simulink model "BEV_Thermal_Management"  (R2025a)
settings: Solver=ode23t  StartTime=0  StopTime=765  MaxStep=5  RelTol=1e-3  AbsTol=1e-3
model workspace: external: MATLAB File BEV_Thermal_Management_param.m (data not in the file)
undefined symbols (not defined in the file): Battery, bulb, cabin_doors_conductivity, cabin_duct_area, cabin_glass_conductivity, cabin_roof_conductivity, cabin_T_init, chiller_area_primary, chiller_N_baffles, chiller_N_tubes, chiller_tube_D, chiller_tube_L, chiller_wall_conductivity, chiller_wall_thickness, compressor_rpm_LUT, condenser_air_area_flow, condenser_air_area_primary, condenser_W, condenser_wall_conductivity, condenser_wall_thickness, coolant_channel_D, coolant_pipe_area, coolant_pipe_D, coolant_T_init, coolant_tank_area, coolant_tank_volume, coolant_valve_D_ratio_max, coolant_valve_D_ratio_min, coolant_valve_displacement, coolant_valve_S_max, cycle, DCDC, Edrive, evaporator_air_area_flow, evaporator_air_area_primary, evaporator_W, evaporator_wall_conductivity, evaporator_wall_thickness, heater_max_power, ModuleType1, outlet, ptc_max_power, pump_speed_max, radiationReflectionShields, radiator_air_area_flow, radiator_air_area_primary, radiator_W, radiator_wall_conductivity, radiator_wall_thickness, refrigerant_alpha_init, refrigerant_pipe_D, transRatio
libraries: fl_lib x264, nesl_utility x91, SimscapeFluids_lib x22, sdl_lib x13, ee_lib x9, nesl_utility_internal x4, slpidlib x3, BatteryProtection x3, batt_lib x2, BatteryCurrentManagement x1, autolibsharedcommon x1, simulink x1
(part 8 of 9)

== system BEV_Thermal_Management/Evaporator/SR5 ==
  Absolute Reference (2P) : fl_lib/Two-Phase Fluid/Elements/Absolute Reference (2P)
  Mass & Energy Flow Rate Sensor (2P) : fl_lib/Two-Phase Fluid/Sensors/Flow Rate Sensor (2P)  mass_flow_measure=true  volumetric_flow_measure=false  energy_flow_measure=true
      settings: InternalSimscapePortConfiguration="{\"Bottom\":[{\"id\":\"PHI\",\"label\":\"φ\",\"type\":\"output\"}],\"Left\":[{\"id\":\"A\",\"label\":\"A\",\"type\":\"foundation.two_phase_fluid.two_phase_fluid\"}],\"Right\":[{\"id\":\"B\",\"label\":\"B\",\"type\":\"foundation.two_phase_fluid.two_phase_fluid\"},{\"id\":\"M\",\"label\":\"M\",\"type\":\"output\"}],\"Top\":[]}"
  PS-Simulink Converter : nesl_utility/PS-Simulink Converter  PhysicalDomain=network_engine_domain  SubClassName=ps_output  LeftPortType=input  RightPortType=output  PseudoPeriodic=off  Frequencies=[]  VectorFormat=1-D array  Unit=W  AffineConversion=off
  PS-Simulink Converter1 : nesl_utility/PS-Simulink Converter  PhysicalDomain=network_engine_domain  SubClassName=ps_output  LeftPortType=input  RightPortType=output  PseudoPeriodic=off  Frequencies=[]  VectorFormat=inherit  Unit=degC  AffineConversion=off
  Pressure & Internal Energy Sensor (2P) : fl_lib/Two-Phase Fluid/Sensors/Pressure, Temperature & Internal Energy Sensor (2P)  reference=foundation.enum.MeasurementReference.difference  pressure=true  pressure_spec=foundation.enum.PressureMeasementSpec.Absolute  temperature=false  internal_energy=true
      settings: InternalSimscapePortConfiguration="{\"Bottom\":[{\"id\":\"U\",\"label\":\"U\",\"type\":\"output\"}],\"Left\":[{\"id\":\"A\",\"label\":\"A\",\"type\":\"foundation.two_phase_fluid.two_phase_fluid\"}],\"Right\":[{\"id\":\"B\",\"label\":\"B\",\"type\":\"foundation.two_phase_fluid.two_phase_fluid\"},{\"id\":\"P\",\"label\":\"P\",\"type\":\"output\"}],\"Top\":[]}"
  Terminator : Terminator
  Thermodynamic Properties Sensor (2P)1 : fl_lib/Two-Phase Fluid/Sensors/Thermodynamic Properties Sensor (2P)  temperature=true  enthalpy=true  density=false  specific_volume=true  entropy=true
      settings: InternalSimscapePortConfiguration="{\"Bottom\":[{\"id\":\"V\",\"label\":\"v\",\"type\":\"output\"},{\"id\":\"S\",\"label\":\"s\",\"type\":\"output\"}],\"Left\":[{\"id\":\"A\",\"label\":\"A\",\"type\":\"foundation.two_phase_fluid.two_phase_fluid\"}],\"Right\":[{\"id\":\"T\",\"label\":\"T\",\"type\":\"output\"},{\"id\":\"H\",\"label\":\"h\",\"type\":\"output\"}],\"Top\":[]}"
  B : PMIOPort  Side=Left
  A : PMIOPort  Port=2  Side=Right
  tag scope: Phi_evap_in=global
  wires:
  PS-Simulink Converter/1 -> [Phi_evap_in]
  PS-Simulink Converter1/1 -> Terminator/1  "tempRefEvapIn"
  connections:
  B/RConn1 -- Mass & Energy Flow Rate Sensor (2P)/RConn1
  Mass & Energy Flow Rate Sensor (2P)/LConn1 -- Thermodynamic Properties Sensor (2P)1/LConn1 -- Pressure & Internal Energy Sensor (2P)/LConn1 -- A/RConn1
  Mass & Energy Flow Rate Sensor (2P)/RConn3 -- PS-Simulink Converter/LConn1
  Absolute Reference (2P)/LConn1 -- Pressure & Internal Energy Sensor (2P)/RConn1
  PS-Simulink Converter1/LConn1 -- Thermodynamic Properties Sensor (2P)1/RConn1

== system BEV_Thermal_Management/Evaporator/SR6 ==
  Absolute Reference (2P) : fl_lib/Two-Phase Fluid/Elements/Absolute Reference (2P)
  Mass & Energy Flow Rate Sensor (2P) : fl_lib/Two-Phase Fluid/Sensors/Flow Rate Sensor (2P)  mass_flow_measure=true  volumetric_flow_measure=false  energy_flow_measure=true
      settings: InternalSimscapePortConfiguration="{\"Bottom\":[{\"id\":\"PHI\",\"label\":\"φ\",\"type\":\"output\"}],\"Left\":[{\"id\":\"A\",\"label\":\"A\",\"type\":\"foundation.two_phase_fluid.two_phase_fluid\"}],\"Right\":[{\"id\":\"B\",\"label\":\"B\",\"type\":\"foundation.two_phase_fluid.two_phase_fluid\"},{\"id\":\"M\",\"label\":\"M\",\"type\":\"output\"}],\"Top\":[]}"
  PS-Simulink Converter : nesl_utility/PS-Simulink Converter  PhysicalDomain=network_engine_domain  SubClassName=ps_output  LeftPortType=input  RightPortType=output  PseudoPeriodic=off  Frequencies=[]  VectorFormat=1-D array  Unit=W  AffineConversion=off
  PS-Simulink Converter1 : nesl_utility/PS-Simulink Converter  PhysicalDomain=network_engine_domain  SubClassName=ps_output  LeftPortType=input  RightPortType=output  PseudoPeriodic=off  Frequencies=[]  VectorFormat=1-D array  Unit=MPa  AffineConversion=off
  PS-Simulink Converter2 : nesl_utility/PS-Simulink Converter  PhysicalDomain=network_engine_domain  SubClassName=ps_output  LeftPortType=input  RightPortType=output  PseudoPeriodic=off  Frequencies=[]  VectorFormat=inherit  Unit=degC  AffineConversion=off
  Pressure & Internal Energy Sensor (2P) : fl_lib/Two-Phase Fluid/Sensors/Pressure, Temperature & Internal Energy Sensor (2P)  reference=foundation.enum.MeasurementReference.difference  pressure=true  pressure_spec=foundation.enum.PressureMeasementSpec.Absolute  temperature=false  internal_energy=true
      settings: InternalSimscapePortConfiguration="{\"Bottom\":[{\"id\":\"U\",\"label\":\"U\",\"type\":\"output\"}],\"Left\":[{\"id\":\"A\",\"label\":\"A\",\"type\":\"foundation.two_phase_fluid.two_phase_fluid\"}],\"Right\":[{\"id\":\"B\",\"label\":\"B\",\"type\":\"foundation.two_phase_fluid.two_phase_fluid\"},{\"id\":\"P\",\"label\":\"P\",\"type\":\"output\"}],\"Top\":[]}"
  Terminator : Terminator
  Thermodynamic Properties Sensor (2P)1 : fl_lib/Two-Phase Fluid/Sensors/Thermodynamic Properties Sensor (2P)  temperature=true  enthalpy=true  density=false  specific_volume=true  entropy=true
      settings: InternalSimscapePortConfiguration="{\"Bottom\":[{\"id\":\"V\",\"label\":\"v\",\"type\":\"output\"},{\"id\":\"S\",\"label\":\"s\",\"type\":\"output\"}],\"Left\":[{\"id\":\"A\",\"label\":\"A\",\"type\":\"foundation.two_phase_fluid.two_phase_fluid\"}],\"Right\":[{\"id\":\"T\",\"label\":\"T\",\"type\":\"output\"},{\"id\":\"H\",\"label\":\"h\",\"type\":\"output\"}],\"Top\":[]}"
  B : PMIOPort  Side=Left
  A : PMIOPort  Port=2  Side=Right
  tag scope: Phi_evap_out=global, p_evap=global
  wires:
  PS-Simulink Converter/1 -> [Phi_evap_out]
  PS-Simulink Converter1/1 -> [p_evap]
  PS-Simulink Converter2/1 -> Terminator/1  "tempRefEvapOut"
  connections:
  B/RConn1 -- Mass & Energy Flow Rate Sensor (2P)/RConn1
  Mass & Energy Flow Rate Sensor (2P)/LConn1 -- Thermodynamic Properties Sensor (2P)1/LConn1 -- Pressure & Internal Energy Sensor (2P)/LConn1 -- A/RConn1
  Mass & Energy Flow Rate Sensor (2P)/RConn3 -- PS-Simulink Converter/LConn1
  Absolute Reference (2P)/LConn1 -- Pressure & Internal Energy Sensor (2P)/RConn1
  PS-Simulink Converter1/LConn1 -- Pressure & Internal Energy Sensor (2P)/RConn2
  PS-Simulink Converter2/LConn1 -- Thermodynamic Properties Sensor (2P)1/RConn1

== system BEV_Thermal_Management/Heater/Current calculator ==
  Controlled Current Source : fl_lib/Electrical/Electrical Sources/Controlled Current Source
  Electrical Reference : fl_lib/Electrical/Electrical Elements/Electrical Reference
  Electrical Reference1 : fl_lib/Electrical/Electrical Elements/Electrical Reference
  PS Divide : fl_lib/Physical Signals/Functions/PS Divide
  Voltage Sensor : fl_lib/Electrical/Electrical Sensors/Voltage Sensor
  Conn2 : PMIOPort  Side=Left
  Conn1 : PMIOPort  Port=2  Side=Left
  connections:
  Electrical Reference/LConn1 -- Controlled Current Source/LConn1
  Controlled Current Source/RConn2 -- Voltage Sensor/LConn1 -- Conn2/RConn1
  PS Divide/LConn1 -- Conn1/RConn1
  Voltage Sensor/RConn2 -- Electrical Reference1/LConn1
  Controlled Current Source/RConn1 -- PS Divide/RConn1
  Voltage Sensor/RConn1 -- PS Divide/LConn2

== system BEV_Thermal_Management/Heater/SC1 ==
  Absolute Reference (TL) : fl_lib/Thermal Liquid/Elements/Absolute Reference (TL)
  PS-Simulink Converter1 : nesl_utility/PS-Simulink Converter  PhysicalDomain=network_engine_domain  SubClassName=ps_output  LeftPortType=input  RightPortType=output  PseudoPeriodic=off  Frequencies=[]  VectorFormat=inherit  Unit=degC  AffineConversion=on
  Pressure & Temperature Sensor (TL) : fl_lib/Thermal Liquid/Sensors/Pressure & Temperature Sensor (TL)  reference=foundation.enum.MeasurementReference.difference  pressure=true  pressure_spec=foundation.enum.PressureMeasementSpec.Absolute  temperature=true
      settings: InternalSimscapePortConfiguration="{\"Bottom\":[{\"id\":\"T\",\"label\":\"T\",\"type\":\"output\"}],\"Left\":[{\"id\":\"A\",\"label\":\"A\",\"type\":\"foundation.thermal_liquid.thermal_liquid\"}],\"Right\":[{\"id\":\"B\",\"label\":\"B\",\"type\":\"foundation.thermal_liquid.thermal_liquid\"},{\"id\":\"P\",\"label\":\"P\",\"type\":\"output\"}],\"Top\":[]}"
  Terminator : Terminator
  B : PMIOPort  Side=Left
  A : PMIOPort  Port=2  Side=Right
  wires:
  PS-Simulink Converter1/1 -> Terminator/1  "tempCoolHeaterOut"
  connections:
  Pressure & Temperature Sensor (TL)/LConn1 -- A/RConn1 -- B/RConn1
  Absolute Reference (TL)/LConn1 -- Pressure & Temperature Sensor (TL)/RConn1
  PS-Simulink Converter1/LConn1 -- Pressure & Temperature Sensor (TL)/RConn3

== system BEV_Thermal_Management/Heater/SC7 ==
  Absolute Reference (TL) : fl_lib/Thermal Liquid/Elements/Absolute Reference (TL)
  PS-Simulink Converter1 : nesl_utility/PS-Simulink Converter  PhysicalDomain=network_engine_domain  SubClassName=ps_output  LeftPortType=input  RightPortType=output  PseudoPeriodic=off  Frequencies=[]  VectorFormat=inherit  Unit=degC  AffineConversion=on
  Pressure & Temperature Sensor (TL) : fl_lib/Thermal Liquid/Sensors/Pressure & Temperature Sensor (TL)  reference=foundation.enum.MeasurementReference.difference  pressure=true  pressure_spec=foundation.enum.PressureMeasementSpec.Absolute  temperature=true
      settings: InternalSimscapePortConfiguration="{\"Bottom\":[{\"id\":\"T\",\"label\":\"T\",\"type\":\"output\"}],\"Left\":[{\"id\":\"A\",\"label\":\"A\",\"type\":\"foundation.thermal_liquid.thermal_liquid\"}],\"Right\":[{\"id\":\"B\",\"label\":\"B\",\"type\":\"foundation.thermal_liquid.thermal_liquid\"},{\"id\":\"P\",\"label\":\"P\",\"type\":\"output\"}],\"Top\":[]}"
  Terminator : Terminator
  B : PMIOPort  Side=Left
  A : PMIOPort  Port=2  Side=Right
  wires:
  PS-Simulink Converter1/1 -> Terminator/1  "tempCoolHeaterIn"
  connections:
  Pressure & Temperature Sensor (TL)/LConn1 -- A/RConn1 -- B/RConn1
  Absolute Reference (TL)/LConn1 -- Pressure & Temperature Sensor (TL)/RConn1
  PS-Simulink Converter1/LConn1 -- Pressure & Temperature Sensor (TL)/RConn3

== system BEV_Thermal_Management/Motor/PWRS3 ==
  Electrical Reference : fl_lib/Electrical/Electrical Elements/Electrical Reference
  PS Terminator : fl_lib/Physical Signals/Sinks/PS Terminator
  Power Sensor : ee_lib/Sensors & Transducers/Power Sensor  measurement_type=1  averaging_period=1e-4 s
  HV : PMIOPort  Side=Left
  EM : PMIOPort  Port=2  Side=Right
  connections:
  Power Sensor/LConn1 -- HV/RConn1
  Power Sensor/LConn2 -- EM/RConn1
  Power Sensor/LConn3 -- Electrical Reference/LConn1
  PS Terminator/LConn1 -- Power Sensor/RConn1

== system BEV_Thermal_Management/Motor/PWRS4 ==
  Mechanical Rotational Reference : fl_lib/Mechanical/Rotational Elements/Mechanical Rotational Reference
  PS Terminator : fl_lib/Physical Signals/Sinks/PS Terminator
  Power : sdl_lib/Sensors/Rotational Power Sensor  measurement_type=sdl.enum.rotationalPowerSensorType.instantaneous  averaging_period=1 s  max_frequency=1000 Hz  max_speed=1000 rpm
      settings: InternalSimscapePortConfiguration="{\"Bottom\":[],\"Left\":[{\"id\":\"S\",\"label\":\"S\",\"type\":\"foundation.mechanical.rotational.rotational\"},{\"id\":\"R\",\"label\":\"R\",\"type\":\"foundation.mechanical.rotational.rotational\"},{\"id\":\"C\",\"label\":\"C\",\"type\":\"foundation.mechanical.rotational.rotational\"}],\"Right\":[{\"id\":\"P\",\"label\":\"P\",\"type\":\"output\"}],\"Top\":[]}"
  C : PMIOPort  Side=Left
  B : PMIOPort  Port=2  Side=Right
  connections:
  Power/LConn1 -- C/RConn1
  Power/LConn3 -- Mechanical Rotational Reference/LConn1
  B/RConn1 -- Power/LConn2
  Power/RConn1 -- PS Terminator/LConn1

== system BEV_Thermal_Management/Motor/PWRS5 ==
  Mechanical Rotational Reference : fl_lib/Mechanical/Rotational Elements/Mechanical Rotational Reference
  PS Terminator : fl_lib/Physical Signals/Sinks/PS Terminator
  Power : sdl_lib/Sensors/Rotational Power Sensor  measurement_type=sdl.enum.rotationalPowerSensorType.instantaneous  averaging_period=1 s  max_frequency=1000 Hz  max_speed=1000 rpm
      settings: InternalSimscapePortConfiguration="{\"Bottom\":[],\"Left\":[{\"id\":\"S\",\"label\":\"S\",\"type\":\"foundation.mechanical.rotational.rotational\"},{\"id\":\"R\",\"label\":\"R\",\"type\":\"foundation.mechanical.rotational.rotational\"},{\"id\":\"C\",\"label\":\"C\",\"type\":\"foundation.mechanical.rotational.rotational\"}],\"Right\":[{\"id\":\"P\",\"label\":\"P\",\"type\":\"output\"}],\"Top\":[]}"
  F : PMIOPort  Side=Left
  RA : PMIOPort  Port=2  Side=Right
  connections:
  Power/LConn1 -- F/RConn1
  Power/LConn3 -- Mechanical Rotational Reference/LConn1
  RA/RConn1 -- Power/LConn2
  Power/RConn1 -- PS Terminator/LConn1

== system BEV_Thermal_Management/Motor/SC5 ==
  Absolute Reference (TL) : fl_lib/Thermal Liquid/Elements/Absolute Reference (TL)
  Mass & Energy Flow Rate Sensor (TL) : fl_lib/Thermal Liquid/Sensors/Flow Rate Sensor (TL)  mass_flow_measure=true  volumetric_flow_measure=false  energy_flow_measure=true
      settings: InternalSimscapePortConfiguration="{\"Bottom\":[{\"id\":\"PHI\",\"label\":\"φ\",\"type\":\"output\"}],\"Left\":[{\"id\":\"A\",\"label\":\"A\",\"type\":\"foundation.thermal_liquid.thermal_liquid\"}],\"Right\":[{\"id\":\"B\",\"label\":\"B\",\"type\":\"foundation.thermal_liquid.thermal_liquid\"},{\"id\":\"M\",\"label\":\"M\",\"type\":\"output\"}],\"Top\":[]}"
  PS-Simulink Converter : nesl_utility/PS-Simulink Converter  PhysicalDomain=network_engine_domain  SubClassName=ps_output  LeftPortType=input  RightPortType=output  PseudoPeriodic=off  Frequencies=[]  VectorFormat=1-D array  Unit=W  AffineConversion=off
  PS-Simulink Converter1 : nesl_utility/PS-Simulink Converter  PhysicalDomain=network_engine_domain  SubClassName=ps_output  LeftPortType=input  RightPortType=output  PseudoPeriodic=off  Frequencies=[]  VectorFormat=inherit  Unit=degC  AffineConversion=on
  Pressure & Temperature Sensor (TL) : fl_lib/Thermal Liquid/Sensors/Pressure & Temperature Sensor (TL)  reference=foundation.enum.MeasurementReference.difference  pressure=true  pressure_spec=foundation.enum.PressureMeasementSpec.Absolute  temperature=true
      settings: InternalSimscapePortConfiguration="{\"Bottom\":[{\"id\":\"T\",\"label\":\"T\",\"type\":\"output\"}],\"Left\":[{\"id\":\"A\",\"label\":\"A\",\"type\":\"foundation.thermal_liquid.thermal_liquid\"}],\"Right\":[{\"id\":\"B\",\"label\":\"B\",\"type\":\"foundation.thermal_liquid.thermal_liquid\"},{\"id\":\"P\",\"label\":\"P\",\"type\":\"output\"}],\"Top\":[]}"
  Terminator : Terminator
  A : PMIOPort  Side=Left
  B : PMIOPort  Port=2  Side=Right
  tag scope: Phi_motor_in=global
  wires:
  PS-Simulink Converter/1 -> [Phi_motor_in]
  PS-Simulink Converter1/1 -> Terminator/1  "tempCoolEMIn"
  connections:
  Pressure & Temperature Sensor (TL)/LConn1 -- A/RConn1 -- Mass & Energy Flow Rate Sensor (TL)/LConn1
  Mass & Energy Flow Rate Sensor (TL)/RConn1 -- B/RConn1
  Absolute Reference (TL)/LConn1 -- Pressure & Temperature Sensor (TL)/RConn1
  Mass & Energy Flow Rate Sensor (TL)/RConn3 -- PS-Simulink Converter/LConn1
  PS-Simulink Converter1/LConn1 -- Pressure & Temperature Sensor (TL)/RConn3

== system BEV_Thermal_Management/Motor/SC6 ==
  Absolute Reference (TL) : fl_lib/Thermal Liquid/Elements/Absolute Reference (TL)
  Mass & Energy Flow Rate Sensor (TL) : fl_lib/Thermal Liquid/Sensors/Flow Rate Sensor (TL)  mass_flow_measure=true  volumetric_flow_measure=false  energy_flow_measure=true
      settings: InternalSimscapePortConfiguration="{\"Bottom\":[{\"id\":\"PHI\",\"label\":\"φ\",\"type\":\"output\"}],\"Left\":[{\"id\":\"A\",\"label\":\"A\",\"type\":\"foundation.thermal_liquid.thermal_liquid\"}],\"Right\":[{\"id\":\"B\",\"label\":\"B\",\"type\":\"foundation.thermal_liquid.thermal_liquid\"},{\"id\":\"M\",\"label\":\"M\",\"type\":\"output\"}],\"Top\":[]}"
  PS-Simulink Converter : nesl_utility/PS-Simulink Converter  PhysicalDomain=network_engine_domain  SubClassName=ps_output  LeftPortType=input  RightPortType=output  PseudoPeriodic=off  Frequencies=[]  VectorFormat=1-D array  Unit=W  AffineConversion=off
  PS-Simulink Converter1 : nesl_utility/PS-Simulink Converter  PhysicalDomain=network_engine_domain  SubClassName=ps_output  LeftPortType=input  RightPortType=output  PseudoPeriodic=off  Frequencies=[]  VectorFormat=1-D array  Unit=degC  AffineConversion=on
  PS-Simulink Converter2 : nesl_utility/PS-Simulink Converter  PhysicalDomain=network_engine_domain  SubClassName=ps_output  LeftPortType=input  RightPortType=output  PseudoPeriodic=off  Frequencies=[]  VectorFormat=inherit  Unit=kg/s  AffineConversion=off
  Pressure & Temperature Sensor (TL) : fl_lib/Thermal Liquid/Sensors/Pressure & Temperature Sensor (TL)  reference=foundation.enum.MeasurementReference.difference  pressure=true  pressure_spec=foundation.enum.PressureMeasementSpec.Absolute  temperature=true
      settings: InternalSimscapePortConfiguration="{\"Bottom\":[{\"id\":\"T\",\"label\":\"T\",\"type\":\"output\"}],\"Left\":[{\"id\":\"A\",\"label\":\"A\",\"type\":\"foundation.thermal_liquid.thermal_liquid\"}],\"Right\":[{\"id\":\"B\",\"label\":\"B\",\"type\":\"foundation.thermal_liquid.thermal_liquid\"},{\"id\":\"P\",\"label\":\"P\",\"type\":\"output\"}],\"Top\":[]}"
  Terminator : Terminator
  A : PMIOPort  Side=Left
  B : PMIOPort  Port=2  Side=Right
  tag scope: Phi_motor_out=global, T_coolant_motor_out=global
  wires:
  PS-Simulink Converter/1 -> [Phi_motor_out]
  PS-Simulink Converter1/1 -> [T_coolant_motor_out]  "tempCoolEMOut"
  PS-Simulink Converter2/1 -> Terminator/1  "tempCoolEMOut"
  connections:
  Pressure & Temperature Sensor (TL)/LConn1 -- A/RConn1 -- Mass & Energy Flow Rate Sensor (TL)/LConn1
  Mass & Energy Flow Rate Sensor (TL)/RConn1 -- B/RConn1
  Absolute Reference (TL)/LConn1 -- Pressure & Temperature Sensor (TL)/RConn1
  Mass & Energy Flow Rate Sensor (TL)/RConn3 -- PS-Simulink Converter/LConn1
  PS-Simulink Converter1/LConn1 -- Pressure & Temperature Sensor (TL)/RConn3
  PS-Simulink Converter2/LConn1 -- Mass & Energy Flow Rate Sensor (TL)/RConn2

== system BEV_Thermal_Management/Motor Pump/Power sensor ==
  MRR3 : fl_lib/Mechanical/Rotational Elements/Mechanical Rotational Reference
  Pump power : fl_lib/Physical Signals/Functions/PS Product
  Rotational Motion Sensor : fl_lib/Mechanical/Mechanical Sensors/Ideal Rotational Motion Sensor  reference=foundation.enum.MeasurementReference.difference  acceleration_port=false  velocity_port=true  position_port=true  wrap_angle=simscape.enum.onoff.off  offset=0 rad
  Torque Sensor : fl_lib/Mechanical/Mechanical Sensors/Ideal Torque Sensor
  A : PMIOPort  Side=Left
  P : PMIOPort  Port=2  Side=Left
  B : PMIOPort  Port=3  Side=Right
  connections:
  Torque Sensor/RConn2 -- Pump power/LConn1
  Torque Sensor/RConn1 -- B/RConn1
  Rotational Motion Sensor/LConn1 -- Torque Sensor/LConn1 -- A/RConn1
  Rotational Motion Sensor/RConn2 -- Pump power/LConn2
  MRR3/LConn1 -- Rotational Motion Sensor/RConn1
  Pump power/RConn1 -- P/RConn1

== system BEV_Thermal_Management/PTC/Current calculator ==
  Controlled Current Source : fl_lib/Electrical/Electrical Sources/Controlled Current Source
  Electrical Reference : fl_lib/Electrical/Electrical Elements/Electrical Reference
  Electrical Reference1 : fl_lib/Electrical/Electrical Elements/Electrical Reference
  PS Divide : fl_lib/Physical Signals/Functions/PS Divide
  Voltage Sensor : fl_lib/Electrical/Electrical Sensors/Voltage Sensor
  Conn2 : PMIOPort  Side=Left
  Conn1 : PMIOPort  Port=2  Side=Left
  connections:
  Electrical Reference/LConn1 -- Controlled Current Source/LConn1
  Controlled Current Source/RConn2 -- Conn2/RConn1 -- Voltage Sensor/LConn1
  PS Divide/LConn1 -- Conn1/RConn1
  Voltage Sensor/RConn2 -- Electrical Reference1/LConn1
  Controlled Current Source/RConn1 -- PS Divide/RConn1
  Voltage Sensor/RConn1 -- PS Divide/LConn2

== system BEV_Thermal_Management/Parallel-Serial Mode Valve/Battery Coolant Tank Heat Transfer ==
  Convective Heat Transfer : fl_lib/Thermal/Thermal Elements/Convective Heat Transfer  thermal_type=foundation.enum.constant_variable.constant  area=3 * coolant_tank_area m^2  heat_tr_coeff=20 W/(m^2 * K)  min_heat_tr_coeff=1e-3 W/(K*m^2)  T_specify=off  T_priority=None  T=0 K  T_nominal_specify=off  T_nominal_value=1  T_nominal_unit=K  Q_specify=off  Q_priority=None  Q=0 W  Q_nominal_specify=off  Q_nominal_value=1  Q_nominal_unit=W
  Convective Heat Transfer1 : fl_lib/Thermal/Thermal Elements/Convective Heat Transfer  thermal_type=foundation.enum.constant_variable.constant  area=3 * coolant_tank_area m^2  heat_tr_coeff=20 W/(m^2 * K)  min_heat_tr_coeff=1e-3 W/(K*m^2)  T_specify=off  T_priority=None  T=0 K  T_nominal_specify=off  T_nominal_value=1  T_nominal_unit=K  Q_specify=off  Q_priority=None  Q=0 W  Q_nominal_specify=off  Q_nominal_value=1  Q_nominal_unit=W
  Environment Temperature : fl_lib/Thermal/Thermal Sources/Controlled Temperature Source
  Simulink-PS Converter : nesl_utility/Simulink-PS Converter  PhysicalDomain=network_engine_domain  SubClassName=ps_input  LeftPortType=input  RightPortType=output  PseudoPeriodic=off  Frequencies=[]  NoiseDistribution=none  NoiseParameters=[]  Unit=degC  AffineConversion=on  FilteringAndDerivatives=provide  SimscapeFilterOrder=1  InputFilterTimeConstant=0.001  UdotUserProvided=0
  Thermal Reference : fl_lib/Thermal/Thermal Elements/Thermal Reference
  A : PMIOPort  Side=Left
  B : PMIOPort  Port=2  Side=Left
  wires:
  [T_env] -> Simulink-PS Converter/1
  connections:
  Environment Temperature/LConn1 -- Convective Heat Transfer/RConn1 -- Convective Heat Transfer1/RConn1
  Thermal Reference/LConn1 -- Environment Temperature/RConn2
  Simulink-PS Converter/RConn1 -- Environment Temperature/RConn1
  B/RConn1 -- Convective Heat Transfer1/LConn1
  Convective Heat Transfer/LConn1 -- A/RConn1

== system BEV_Thermal_Management/Parallel-Serial Mode Valve/Motor Coolant Tank Heat Transfer ==
  Convective Heat Transfer : fl_lib/Thermal/Thermal Elements/Convective Heat Transfer  thermal_type=foundation.enum.constant_variable.constant  area=3 * coolant_tank_area m^2  heat_tr_coeff=20 W/(m^2 * K)  min_heat_tr_coeff=1e-3 W/(K*m^2)  T_specify=off  T_priority=None  T=0 K  T_nominal_specify=off  T_nominal_value=1  T_nominal_unit=K  Q_specify=off  Q_priority=None  Q=0 W  Q_nominal_specify=off  Q_nominal_value=1  Q_nominal_unit=W
  Convective Heat Transfer1 : fl_lib/Thermal/Thermal Elements/Convective Heat Transfer  thermal_type=foundation.enum.constant_variable.constant  area=3 * coolant_tank_area m^2  heat_tr_coeff=20 W/(m^2 * K)  min_heat_tr_coeff=1e-3 W/(K*m^2)  T_specify=off  T_priority=None  T=0 K  T_nominal_specify=off  T_nominal_value=1  T_nominal_unit=K  Q_specify=off  Q_priority=None  Q=0 W  Q_nominal_specify=off  Q_nominal_value=1  Q_nominal_unit=W
  Environment Temperature : fl_lib/Thermal/Thermal Sources/Controlled Temperature Source
  Simulink-PS Converter : nesl_utility/Simulink-PS Converter  PhysicalDomain=network_engine_domain  SubClassName=ps_input  LeftPortType=input  RightPortType=output  PseudoPeriodic=off  Frequencies=[]  NoiseDistribution=none  NoiseParameters=[]  Unit=degC  AffineConversion=on  FilteringAndDerivatives=provide  SimscapeFilterOrder=1  InputFilterTimeConstant=0.001  UdotUserProvided=0
  Thermal Reference : fl_lib/Thermal/Thermal Elements/Thermal Reference
  A : PMIOPort  Side=Right
  B : PMIOPort  Port=2  Side=Right
  wires:
  [T_env] -> Simulink-PS Converter/1
  connections:
  Simulink-PS Converter/RConn1 -- Environment Temperature/RConn1
  Thermal Reference/LConn1 -- Environment Temperature/RConn2
  Convective Heat Transfer/RConn1 -- Environment Temperature/LConn1 -- Convective Heat Transfer1/RConn1
  B/RConn1 -- Convective Heat Transfer1/LConn1
  A/RConn1 -- Convective Heat Transfer/LConn1

== system BEV_Thermal_Management/Radiator/Ram Pressure ==
  1/2 : fl_lib/Physical Signals/Functions/PS Gain  gain=0.5
  Controlled Pressure Source (MA) : fl_lib/Moist Air/Sources/Pressure Source (MA)  source_type=foundation.enum.constant_controlled.controlled  pressure_differential=0 MPa  power_spec=foundation.enum.power_spec.isentropic  area_A=cabin_duct_area m^2  area_B=cabin_duct_area m^2
      settings: InternalSimscapePortConfiguration="{\"Bottom\":[],\"Left\":[{\"id\":\"A\",\"label\":\"A\",\"type\":\"foundation.moist_air.moist_air\"},{\"id\":\"P\",\"label\":\"P\",\"type\":\"input\"}],\"Right\":[{\"id\":\"B\",\"label\":\"B\",\"type\":\"foundation.moist_air.moist_air\"}],\"Top\":[]}"
  PS Product : fl_lib/Physical Signals/Functions/PS Product
  Thermodynamic Properties Sensor (MA) : fl_lib/Moist Air/Sensors/Thermodynamic Properties Sensor (MA)  measurement_mass_spec=foundation.enum.measurement_mass_spec.mixture  enthalpy=true  enthalpy_reference=foundation.enum.EnthalpyReference.PropertyTables  density=true  specific_heat=true  entropy=true
      settings: InternalSimscapePortConfiguration="{\"Bottom\":[{\"id\":\"CP\",\"label\":\"cp\",\"type\":\"output\"},{\"id\":\"S\",\"label\":\"s\",\"type\":\"output\"}],\"Left\":[{\"id\":\"A\",\"label\":\"A\",\"type\":\"foundation.moist_air.moist_air\"}],\"Right\":[{\"id\":\"H\",\"label\":\"h\",\"type\":\"output\"},{\"id\":\"RHO\",\"label\":\"ρ\",\"type\":\"output\"}],\"Top\":[]}"
  sqr : fl_lib/Physical Signals/Functions/PS Math Function  fcn_choice=foundation.enum.math_function.square  v=1
  A : PMIOPort  Side=Left
  V : PMIOPort  Port=2  Side=Left
  B : PMIOPort  Port=3  Side=Right
  connections:
  Controlled Pressure Source (MA)/RConn1 -- B/RConn1
  Controlled Pressure Source (MA)/LConn1 -- Thermodynamic Properties Sensor (MA)/LConn1 -- A/RConn1
  PS Product/RConn1 -- Controlled Pressure Source (MA)/LConn2
  1/2/RConn1 -- PS Product/LConn1
  sqr/RConn1 -- 1/2/LConn1
  V/RConn1 -- sqr/LConn1
  PS Product/LConn2 -- Thermodynamic Properties Sensor (MA)/RConn2

== system BEV_Thermal_Management/Radiator/SC1 ==
  Absolute Reference (TL) : fl_lib/Thermal Liquid/Elements/Absolute Reference (TL)
  Mass & Energy Flow Rate Sensor (TL) : fl_lib/Thermal Liquid/Sensors/Flow Rate Sensor (TL)  mass_flow_measure=true  volumetric_flow_measure=false  energy_flow_measure=true
      settings: InternalSimscapePortConfiguration="{\"Bottom\":[{\"id\":\"PHI\",\"label\":\"φ\",\"type\":\"output\"}],\"Left\":[{\"id\":\"A\",\"label\":\"A\",\"type\":\"foundation.thermal_liquid.thermal_liquid\"}],\"Right\":[{\"id\":\"B\",\"label\":\"B\",\"type\":\"foundation.thermal_liquid.thermal_liquid\"},{\"id\":\"M\",\"label\":\"M\",\"type\":\"output\"}],\"Top\":[]}"
  PS-Simulink Converter : nesl_utility/PS-Simulink Converter  PhysicalDomain=network_engine_domain  SubClassName=ps_output  LeftPortType=input  RightPortType=output  PseudoPeriodic=off  Frequencies=[]  VectorFormat=1-D array  Unit=W  AffineConversion=off
  PS-Simulink Converter1 : nesl_utility/PS-Simulink Converter  PhysicalDomain=network_engine_domain  SubClassName=ps_output  LeftPortType=input  RightPortType=output  PseudoPeriodic=off  Frequencies=[]  VectorFormat=inherit  Unit=degC  AffineConversion=on
  Pressure & Temperature Sensor (TL) : fl_lib/Thermal Liquid/Sensors/Pressure & Temperature Sensor (TL)  reference=foundation.enum.MeasurementReference.difference  pressure=true  pressure_spec=foundation.enum.PressureMeasementSpec.Absolute  temperature=true
      settings: InternalSimscapePortConfiguration="{\"Bottom\":[{\"id\":\"T\",\"label\":\"T\",\"type\":\"output\"}],\"Left\":[{\"id\":\"A\",\"label\":\"A\",\"type\":\"foundation.thermal_liquid.thermal_liquid\"}],\"Right\":[{\"id\":\"B\",\"label\":\"B\",\"type\":\"foundation.thermal_liquid.thermal_liquid\"},{\"id\":\"P\",\"label\":\"P\",\"type\":\"output\"}],\"Top\":[]}"
  Terminator : Terminator
  B : PMIOPort  Side=Left
  A : PMIOPort  Port=2  Side=Right
  tag scope: Phi_rad_in=global
  wires:
  PS-Simulink Converter/1 -> [Phi_rad_in]
  PS-Simulink Converter1/1 -> Terminator/1  "tempCoolRadIn"
  connections:
  Pressure & Temperature Sensor (TL)/LConn1 -- A/RConn1 -- Mass & Energy Flow Rate Sensor (TL)/LConn1
  Mass & Energy Flow Rate Sensor (TL)/RConn1 -- B/RConn1
  Absolute Reference (TL)/LConn1 -- Pressure & Temperature Sensor (TL)/RConn1
  Mass & Energy Flow Rate Sensor (TL)/RConn3 -- PS-Simulink Converter/LConn1
  PS-Simulink Converter1/LConn1 -- Pressure & Temperature Sensor (TL)/RConn3

== system BEV_Thermal_Management/Radiator/SC2 ==
  Absolute Reference (TL) : fl_lib/Thermal Liquid/Elements/Absolute Reference (TL)
  Mass & Energy Flow Rate Sensor (TL) : fl_lib/Thermal Liquid/Sensors/Flow Rate Sensor (TL)  mass_flow_measure=true  volumetric_flow_measure=false  energy_flow_measure=true
      settings: InternalSimscapePortConfiguration="{\"Bottom\":[{\"id\":\"PHI\",\"label\":\"φ\",\"type\":\"output\"}],\"Left\":[{\"id\":\"A\",\"label\":\"A\",\"type\":\"foundation.thermal_liquid.thermal_liquid\"}],\"Right\":[{\"id\":\"B\",\"label\":\"B\",\"type\":\"foundation.thermal_liquid.thermal_liquid\"},{\"id\":\"M\",\"label\":\"M\",\"type\":\"output\"}],\"Top\":[]}"
  PS-Simulink Converter : nesl_utility/PS-Simulink Converter  PhysicalDomain=network_engine_domain  SubClassName=ps_output  LeftPortType=input  RightPortType=output  PseudoPeriodic=off  Frequencies=[]  VectorFormat=1-D array  Unit=W  AffineConversion=off
  PS-Simulink Converter1 : nesl_utility/PS-Simulink Converter  PhysicalDomain=network_engine_domain  SubClassName=ps_output  LeftPortType=input  RightPortType=output  PseudoPeriodic=off  Frequencies=[]  VectorFormat=inherit  Unit=degC  AffineConversion=on
  Pressure & Temperature Sensor (TL) : fl_lib/Thermal Liquid/Sensors/Pressure & Temperature Sensor (TL)  reference=foundation.enum.MeasurementReference.difference  pressure=true  pressure_spec=foundation.enum.PressureMeasementSpec.Absolute  temperature=true
      settings: InternalSimscapePortConfiguration="{\"Bottom\":[{\"id\":\"T\",\"label\":\"T\",\"type\":\"output\"}],\"Left\":[{\"id\":\"A\",\"label\":\"A\",\"type\":\"foundation.thermal_liquid.thermal_liquid\"}],\"Right\":[{\"id\":\"B\",\"label\":\"B\",\"type\":\"foundation.thermal_liquid.thermal_liquid\"},{\"id\":\"P\",\"label\":\"P\",\"type\":\"output\"}],\"Top\":[]}"
  Terminator : Terminator
  B : PMIOPort  Side=Left
  A : PMIOPort  Port=2  Side=Right
  tag scope: Phi_rad_out=global
  wires:
  PS-Simulink Converter/1 -> [Phi_rad_out]
  PS-Simulink Converter1/1 -> Terminator/1  "tempCoolRadOut"
  connections:
  Pressure & Temperature Sensor (TL)/LConn1 -- A/RConn1 -- Mass & Energy Flow Rate Sensor (TL)/LConn1
  Mass & Energy Flow Rate Sensor (TL)/RConn1 -- B/RConn1
  Absolute Reference (TL)/LConn1 -- Pressure & Temperature Sensor (TL)/RConn1
  Mass & Energy Flow Rate Sensor (TL)/RConn3 -- PS-Simulink Converter/LConn1
  PS-Simulink Converter1/LConn1 -- Pressure & Temperature Sensor (TL)/RConn3

== system BEV_Thermal_Management/Scenario/Drive Cycle ==
  Vehicle : Inport
  1-D Lookup Table : Lookup_n-D  NumberOfTableDimensions=1  BreakpointsForDimension1=time  Table=velocity  InternalRulePriority=Speed  RndMeth=Simplest
  1-D Lookup Table1 : Lookup_n-D  NumberOfTableDimensions=1  BreakpointsForDimension1=time  Table=mode  InternalRulePriority=Speed  RndMeth=Simplest
  Clock : Clock
  Scope : Scope  NumInputPorts=4
      settings: ActiveDisplayYMinimum=-14.375  ActiveDisplayYMaximum=109.375
  Stop Simulation : Stop
  Subsystem : Subsystem
  Reference : Outport
  Mode : Outport  Port=2
  wires:
  Subsystem/1(Fault) -> Stop Simulation/1
  Vehicle/1 -> Scope/4, Subsystem/1(VelFdbk)
  1-D Lookup Table/1 -> Reference/1, Scope/1  "Reference"
  Subsystem/3(LowerBnd) -> Scope/3  "Lower Bound"
  Subsystem/2(UpperBnd) -> Scope/2  "Upper Bound"
  Clock/1 -> 1-D Lookup Table/1, 1-D Lookup Table1/1
  1-D Lookup Table1/1 -> Mode/1

== system BEV_Thermal_Management/Battery/Lumped/PWRS1 ==
  Electrical Reference1 : fl_lib/Electrical/Electrical Elements/Electrical Reference
  Power : fl_lib/Physical Signals/Sinks/PS Terminator
  Power Sensor : ee_lib/Sensors & Transducers/Power Sensor  measurement_type=1  averaging_period=1e-4 s
  Batt : PMIOPort  Side=Left
  EM : PMIOPort  Port=2  Side=Right
  connections:
  Power/LConn1 -- Power Sensor/RConn1
  Power Sensor/LConn2 -- EM/RConn1
  Electrical Reference1/LConn1 -- Power Sensor/LConn3
  Power Sensor/LConn1 -- Batt/RConn1

== system BEV_Thermal_Management/Battery/Lumped/SC3 ==
  Absolute Reference (TL) : fl_lib/Thermal Liquid/Elements/Absolute Reference (TL)
  LPIn : fl_lib/Thermal Liquid/Sensors/Thermodynamic Properties Sensor (TL)  internal_energy=true  density=true  specific_heat=true
      settings: InternalSimscapePortConfiguration="{\"Bottom\":[],\"Left\":[{\"id\":\"A\",\"label\":\"A\",\"type\":\"foundation.thermal_liquid.thermal_liquid\"}],\"Right\":[{\"id\":\"U\",\"label\":\"u\",\"type\":\"output\"},{\"id\":\"RHO\",\"label\":\"ρ\",\"type\":\"output\"},{\"id\":\"CP\",\"label\":\"cp\",\"type\":\"output\"}],\"Top\":[]}"
  Mass & Energy Flow Rate Sensor (TL) : fl_lib/Thermal Liquid/Sensors/Flow Rate Sensor (TL)  mass_flow_measure=true  volumetric_flow_measure=false  energy_flow_measure=true
      settings: InternalSimscapePortConfiguration="{\"Bottom\":[{\"id\":\"PHI\",\"label\":\"φ\",\"type\":\"output\"}],\"Left\":[{\"id\":\"A\",\"label\":\"A\",\"type\":\"foundation.thermal_liquid.thermal_liquid\"}],\"Right\":[{\"id\":\"B\",\"label\":\"B\",\"type\":\"foundation.thermal_liquid.thermal_liquid\"},{\"id\":\"M\",\"label\":\"M\",\"type\":\"output\"}],\"Top\":[]}"
  PS-Simulink Converter : nesl_utility/PS-Simulink Converter  PhysicalDomain=network_engine_domain  SubClassName=ps_output  LeftPortType=input  RightPortType=output  PseudoPeriodic=off  Frequencies=[]  VectorFormat=1-D array  Unit=W  AffineConversion=off
  PS-Simulink Converter1 : nesl_utility/PS-Simulink Converter  PhysicalDomain=network_engine_domain  SubClassName=ps_output  LeftPortType=input  RightPortType=output  PseudoPeriodic=off  Frequencies=[]  VectorFormat=1-D array  Unit=degC  AffineConversion=on
  Pressure & Temperature Sensor (TL) : fl_lib/Thermal Liquid/Sensors/Pressure & Temperature Sensor (TL)  reference=foundation.enum.MeasurementReference.difference  pressure=true  pressure_spec=foundation.enum.PressureMeasementSpec.Absolute  temperature=true
      settings: InternalSimscapePortConfiguration="{\"Bottom\":[{\"id\":\"T\",\"label\":\"T\",\"type\":\"output\"}],\"Left\":[{\"id\":\"A\",\"label\":\"A\",\"type\":\"foundation.thermal_liquid.thermal_liquid\"}],\"Right\":[{\"id\":\"B\",\"label\":\"B\",\"type\":\"foundation.thermal_liquid.thermal_liquid\"},{\"id\":\"P\",\"label\":\"P\",\"type\":\"output\"}],\"Top\":[]}"
  B : PMIOPort  Side=Left
  A : PMIOPort  Port=2  Side=Right
  tag scope: Phi_battery_in=global, T_coolant_battery_in=global
  wires:
  PS-Simulink Converter/1 -> [Phi_battery_in]
  PS-Simulink Converter1/1 -> [T_coolant_battery_in]  "tempCoolBattIn"
  connections:
  Pressure & Temperature Sensor (TL)/LConn1 -- LPIn/LConn1 -- A/RConn1 -- Mass & Energy Flow Rate Sensor (TL)/LConn1
  Mass & Energy Flow Rate Sensor (TL)/RConn1 -- B/RConn1
  Absolute Reference (TL)/LConn1 -- Pressure & Temperature Sensor (TL)/RConn1
  Mass & Energy Flow Rate Sensor (TL)/RConn3 -- PS-Simulink Converter/LConn1
  PS-Simulink Converter1/LConn1 -- Pressure & Temperature Sensor (TL)/RConn3

== system BEV_Thermal_Management/Battery/Lumped/SC4 ==
  Absolute Reference (TL) : fl_lib/Thermal Liquid/Elements/Absolute Reference (TL)
  LPOut : fl_lib/Thermal Liquid/Sensors/Thermodynamic Properties Sensor (TL)  internal_energy=true  density=true  specific_heat=true
      settings: InternalSimscapePortConfiguration="{\"Bottom\":[],\"Left\":[{\"id\":\"A\",\"label\":\"A\",\"type\":\"foundation.thermal_liquid.thermal_liquid\"}],\"Right\":[{\"id\":\"U\",\"label\":\"u\",\"type\":\"output\"},{\"id\":\"RHO\",\"label\":\"ρ\",\"type\":\"output\"},{\"id\":\"CP\",\"label\":\"cp\",\"type\":\"output\"}],\"Top\":[]}"
  Mass & Energy Flow Rate Sensor (TL) : fl_lib/Thermal Liquid/Sensors/Flow Rate Sensor (TL)  mass_flow_measure=true  volumetric_flow_measure=false  energy_flow_measure=true
      settings: InternalSimscapePortConfiguration="{\"Bottom\":[{\"id\":\"PHI\",\"label\":\"φ\",\"type\":\"output\"}],\"Left\":[{\"id\":\"A\",\"label\":\"A\",\"type\":\"foundation.thermal_liquid.thermal_liquid\"}],\"Right\":[{\"id\":\"B\",\"label\":\"B\",\"type\":\"foundation.thermal_liquid.thermal_liquid\"},{\"id\":\"M\",\"label\":\"M\",\"type\":\"output\"}],\"Top\":[]}"
  PS-Simulink Converter : nesl_utility/PS-Simulink Converter  PhysicalDomain=network_engine_domain  SubClassName=ps_output  LeftPortType=input  RightPortType=output  PseudoPeriodic=off  Frequencies=[]  VectorFormat=1-D array  Unit=W  AffineConversion=off
  PS-Simulink Converter1 : nesl_utility/PS-Simulink Converter  PhysicalDomain=network_engine_domain  SubClassName=ps_output  LeftPortType=input  RightPortType=output  PseudoPeriodic=off  Frequencies=[]  VectorFormat=inherit  Unit=degC  AffineConversion=on
  Pressure & Temperature Sensor (TL) : fl_lib/Thermal Liquid/Sensors/Pressure & Temperature Sensor (TL)  reference=foundation.enum.MeasurementReference.difference  pressure=true  pressure_spec=foundation.enum.PressureMeasementSpec.Absolute  temperature=true
      settings: InternalSimscapePortConfiguration="{\"Bottom\":[{\"id\":\"T\",\"label\":\"T\",\"type\":\"output\"}],\"Left\":[{\"id\":\"A\",\"label\":\"A\",\"type\":\"foundation.thermal_liquid.thermal_liquid\"}],\"Right\":[{\"id\":\"B\",\"label\":\"B\",\"type\":\"foundation.thermal_liquid.thermal_liquid\"},{\"id\":\"P\",\"label\":\"P\",\"type\":\"output\"}],\"Top\":[]}"
  Terminator : Terminator
  B : PMIOPort  Side=Left
  A : PMIOPort  Port=2  Side=Right
  tag scope: Phi_battery_out=global
  wires:
  PS-Simulink Converter/1 -> [Phi_battery_out]
  PS-Simulink Converter1/1 -> Terminator/1  "tempCoolBattOut"
  connections:
  Pressure & Temperature Sensor (TL)/LConn1 -- LPOut/LConn1 -- A/RConn1 -- Mass & Energy Flow Rate Sensor (TL)/LConn1
  Mass & Energy Flow Rate Sensor (TL)/RConn1 -- B/RConn1
  Absolute Reference (TL)/LConn1 -- Pressure & Temperature Sensor (TL)/RConn1
  Mass & Energy Flow Rate Sensor (TL)/RConn3 -- PS-Simulink Converter/LConn1
  PS-Simulink Converter1/LConn1 -- Pressure & Temperature Sensor (TL)/RConn3

== system BEV_Thermal_Management/Charger/Charger Model/Charger ==
  note: If desired a thermal connection between charger and coolant can be implemented here
  note: Activates charging logic when set to one
  Voltage Cell : Inport
  Charging Logic : Inport  Port=2
  Battery CC-CV : BatteryCurrentManagement/Battery CC-CV  MinMaxFlag=off  MaxCellVoltage=4.0  Kp=100  Ki=10  Kaw=1  Kt=1  Ts=0
      settings: LibrarySourceBlock=batt_sl_lib/Current Management/Battery CC-CV
  Charger : fl_lib/Electrical/Electrical Sources/Controlled Current Source
  Charging with 1.5C : Constant  Value=Battery.Np*Battery.cellAh*1.5
  Electrical Reference : fl_lib/Electrical/Electrical Elements/Electrical Reference
  Ground : Ground
  Simulink-PS Converter1 : nesl_utility/Simulink-PS Converter  PhysicalDomain=network_engine_domain  SubClassName=ps_input  LeftPortType=input  RightPortType=output  PseudoPeriodic=off  Frequencies=[]  NoiseDistribution=none  NoiseParameters=[]  Unit=1  AffineConversion=off  FilteringAndDerivatives=provide  SimscapeFilterOrder=1  InputFilterTimeConstant=0.001  UdotUserProvided=0
  Transfer Fcn1 : TransferFcn  Denominator=[0.1 1]
  A : PMIOPort  Side=Left
  HV : PMIOPort  Port=2  Side=Right
  B : PMIOPort  Port=3  Side=Right
  Battery Charging Current : Outport
  wires:
  Charging with 1.5C/1 -> Battery CC-CV/3
  Voltage Cell/1 -> Battery CC-CV/2
  Transfer Fcn1/1 -> Battery Charging Current/1, Simulink-PS Converter1/1
  Battery CC-CV/1 -> Transfer Fcn1/1
  Charging Logic/1 -> Battery CC-CV/1
  Ground/1 -> Battery CC-CV/4
  connections:
  Electrical Reference/LConn1 -- Charger/RConn2
  B/RConn1 -- A/RConn1
  HV/RConn1 -- Charger/LConn1
  Simulink-PS Converter1/RConn1 -- Charger/RConn1

== system BEV_Thermal_Management/Charger/Charger Model/No Charger ==
  note: If desired a thermal connection between charger and coolant can be implemented here
  Voltage Cell : Inport
  Charging Logic : Inport  Port=2
  Coolant Jacket : SimscapeFluids_lib/Thermal Liquid/Pipes & Fittings/Pipe (TL)  dynamic_compressibility=simscape.enum.onoff.on  inertia=simscape.enum.onoff.off  num_segments=1  pipe_length=0.4 m  cross_section_geometry=fluids.thermal_liquid.pipes_fittings.enum.CrossSectionGeometry.Custom  pipe_diameter=0.1 m  pipe_inner_diameter=0.05 m  pipe_outer_diameter=0.1 m  pipe_width=0.1 m  pipe_height=0.1 m  pipe_major_axis=0.1 m  pipe_minor_axis=0.05 m  pipe_side=0.1 m  pipe_angle=30 deg  area=pi * coolant_channel_D^2 / 4 m^2  Dh=coolant_channel_D m  elevation_spec=foundation.enum.constant_variable.constant  elevation_gain=0 m  gravity_spec=foundation.enum.constant_variable.constant  g=9.81 m/s^2  pressure_loss_spec=fluids.thermal_liquid.pipes_fittings.enum.PressureLossSpec.Haaland  local_pressure_loss_spec=fluids.thermal_liquid.pipes_fittings.enum.LocalLossSpec.AggregateLength  length_add=20 * coolant_channel_D * 4 m  loss_coefficient=0.1  roughness_spec=fluids.thermal_liquid.pipes_fittings.enum.RoughnessSpec.Custom  roughness=1.5e-5 m  Re_friction_TLU=[ 400 1000 1.5e+3 3e+3 4e+3 6e+3 1e+4 2e+4 4e+4 6e+4 1e+5 1e+8 ]  friction_factor_TLU=[ 0.264 0.112 0.07099999999999999 0.0417 0.0387 0.0268 0.025 0.0232 0.0226 0.022 0.0214 0.0214 ]  Re_lam=100  Re_tur=500  shape_factor=64  mdot_nominal=[ 0.1 1 ] kg/s  p_diff_nominal=[ 0.001 0.01 ] MPa  mdot_threshold=1e-6 kg/s  wall_spec=fluids.thermal_liquid.pipes_fittings.enum.wall_spec.rigid  vol_expansion_spec=fluids.thermal_liquid.pipes_fittings.enum.VolumeExpansionSpec.Diameter  area_pressure_gain=1e-6 m^2/MPa  static_pressure_TLU=[.1, 1] MPa  area_pressure_gain_TLU=[1e-05, 1.1e-05] m^2  material_behavior_spec=fluids.thermal_liquid.pipes_fittings.enum.PipeMaterialBehavior.Linear  diameter_pressure_gain=1.2e-6 m/MPa  wall_thickness=0.05 m  elastic_modulus=69 GPa  stress_TLU=[276, 310] MPa  strain_TLU=[.004, .02]  stress_assert_action=simscape.enum.assert.action.none  stress_max=400 MPa  poisson_ratio=0.33  wall_time_constant=0.01 s  thermal_expansion=false  alpha_L_wall=24 um/(deltaK*m)  thermal_expansion_Tref=293.15 K  heat_transfer_spec=fluids.thermal_liquid.pipes_fittings.enum.HeatTransferSpec.DittusBoelter  mdot_nominal_heat=[ 0.1 1 ] kg/s  T_in_nominal=[ 293.15 293.15 ] K  T_out_nominal=[ 300 300 ] K  p_in_nominal_heat=[ 0.101325 0.101325 ] MPa  T_wall_nominal=[ 303.15 303.15 ] K  a_coeff=0.3  b_Re_power=0.8  c_Pr_power=0.33  Nu_lam=3.66  Re_Colburn_TLU=[ 100 150 1000 ]  Colburn_factor_TLU=[ 0.019 0.013 0.002 ]  Re_Nu_TLU=[ 100 150 1000 ]  Pr_Nu_TLU=[ 1 10 ]  Nu_TLU=[ 3.72 4.21; 3.75 4.44; 4.21 7.15 ]  p0_vec=coolant_p_init MPa  T0_vec=coolant_T_init K  mdot0=0.1 kg/s  p_nominal=0.101325 MPa  T_nominal=293.15 K
  Ground1 : Ground
  Terminator : Terminator
  Terminator1 : Terminator
  A : PMIOPort  Side=Left
  HV : PMIOPort  Port=2  Side=Right
  B : PMIOPort  Port=3  Side=Right
  Battery Charging Current : Outport
  wires:
  Ground1/1 -> Battery Charging Current/1
  Charging Logic/1 -> Terminator/1
  Voltage Cell/1 -> Terminator1/1
  connections:
  Coolant Jacket/LConn1 -- A/RConn1
  Coolant Jacket/RConn1 -- B/RConn1

== system BEV_Thermal_Management/Controls/Coolant Loop Control/Battery Heater ==
  T_env : Inport
  T_coolant_battery_in : Inport  Port=2
  Constant : Constant  Value=0
  Relay : Relay  OnSwitchValue=15  OffSwitchValue=5  OnOutputValue=0  OffOutputValue=1  ZeroCross=off
  Switch : Switch  Criteria=u2 > Threshold  Threshold=5  SaturateOnIntegerOverflow=off  InputSameDT=off
  cmd_heater : Outport
  wires:
  T_coolant_battery_in/1 -> Relay/1
  Switch/1 -> cmd_heater/1
  T_env/1 -> Switch/2
  Relay/1 -> Switch/3
  Constant/1 -> Switch/1

== system BEV_Thermal_Management/Controls/Coolant Loop Control/Battery Pump ==
  cmd_motor_pump : Inport
  T_battery : Inport  Port=2
  cmd_chiller_bypass : Inport  Port=3
  parallel_serial : Inport  Port=4
  Constant : Constant  Value=0.3
  Constant1 : Constant  Value=0.5
  MinMax : MinMax  Function=max  Inputs=2
  Relay : Relay  OnSwitchValue=40  OffSwitchValue=35
  Switch : Switch  Criteria=u2 > Threshold  Threshold=0.5  SaturateOnIntegerOverflow=off  InputSameDT=off
  Switch1 : Switch  Criteria=u2 > Threshold  Threshold=0.5  SaturateOnIntegerOverflow=off  InputSameDT=off
  cmd_battery_pump : Outport
  wires:
  T_battery/1 -> Relay/1
  parallel_serial/1 -> Switch/2
  Switch/1 -> cmd_battery_pump/1
  Constant/1 -> Switch1/1
  Constant1/1 -> Switch1/3
  cmd_chiller_bypass/1 -> Switch1/2
  Relay/1 -> MinMax/1
  Switch1/1 -> MinMax/2
  MinMax/1 -> Switch/3
  cmd_motor_pump/1 -> Switch/1

== system BEV_Thermal_Management/Controls/Coolant Loop Control/Chiller Bypass ==
  note: If the temperature of the battery > 35°C, then the chiller is activated
      | If the temperature of the battery < 30°C, then the chiller is bypassed (cmd_chiller_bypass = 1)
  T_battery : Inport
  Relay : Relay  OnSwitchValue=35  OffSwitchValue=30  OnOutputValue=0  OffOutputValue=1
  cmd_chiller_bypass : Outport
  wires:
  Relay/1 -> cmd_chiller_bypass/1
  T_battery/1 -> Relay/1

== system BEV_Thermal_Management/Controls/Coolant Loop Control/Motor Pump ==
  T_motor : Inport
  1-D Lookup Table : Lookup_n-D  NumberOfTableDimensions=1  BreakpointsForDimension1=[-50 45 48 52 58 60 75 130]  IndexSearchMethod=Linear search  BeginIndexSearchUsingPreviousIndexResult=on  Table=[0 0 0.1 0.3 0.5 0.7 1 1]  InternalRulePriority=Speed  RndMeth=Simplest
  Saturation : Saturate  UpperLimit=1  LowerLimit=0.3
  cmd_motor_pump : Outport
  wires:
  T_motor/1 -> 1-D Lookup Table/1
  1-D Lookup Table/1 -> Saturation/1
  Saturation/1 -> cmd_motor_pump/1

== system BEV_Thermal_Management/Controls/Coolant Loop Control/Parallel-Serial Mode ==
  note: If the chiller is active, always switch to parallel mode
  note: In cold weather, the coolant loops are in serial mode so that heat from the motor warms the batteries. If necessary, a heater can provide additional heat.
      |
      | In warm weather, the coolant loops remain in serial mode and both the batteries and the powertrain are cooled by the radiator.
      |
      | In hot weather, the coolant loop switches to parallel mode and separates. One loop cools the powertrain using the radiator. The other cools the batteries using the chiller in the refrigeration loop.
  note: 0 = Parallel mode
      |
      | 1 = Serial mode
  cmd_chiller_bypass : Inport
  T_env : Inport  Port=2
  T_coolant_inverter_out : Inport  Port=3
  Constant : Constant  Value=0
  MinMax : MinMax  Function=max  Inputs=2
  Relay : Relay  OnSwitchValue=40%35  OffSwitchValue=30  OnOutputValue=0  OffOutputValue=1
  Switch : Switch  Criteria=u2 > Threshold  Threshold=0.5  SaturateOnIntegerOverflow=off  InputSameDT=off
  cmd_parallel_serial : Outport
  wires:
  T_env/1 -> MinMax/1
  T_coolant_inverter_out/1 -> MinMax/2
  MinMax/1 -> Relay/1
  Constant/1 -> Switch/3
  Switch/1 -> cmd_parallel_serial/1
  cmd_chiller_bypass/1 -> Switch/2
  Relay/1 -> Switch/1

== system BEV_Thermal_Management/Controls/Coolant Loop Control/Radiator Bypass ==
  note: if T > 35 °C the value is set the valve way to the radiatior is activated -> The systems are cooled down via the radiator
      | if T < 20 °C then the motor, inverter, charger etc. etc. are cooled enough and the radiator is simply bypassed
  T_coolant_inverter_out : Inport
  Relay : Relay  OnSwitchValue=35%25  OffSwitchValue=20  OnOutputValue=0  OffOutputValue=1
  cmd_rad_bypass : Outport
  wires:
  Relay/1 -> cmd_rad_bypass/1
  T_coolant_inverter_out/1 -> Relay/1
